simulink model "smart_irrigation_complete"  (R2026a)
settings: Solver=VariableStepAuto  StopTime=50
libraries: simulink x2

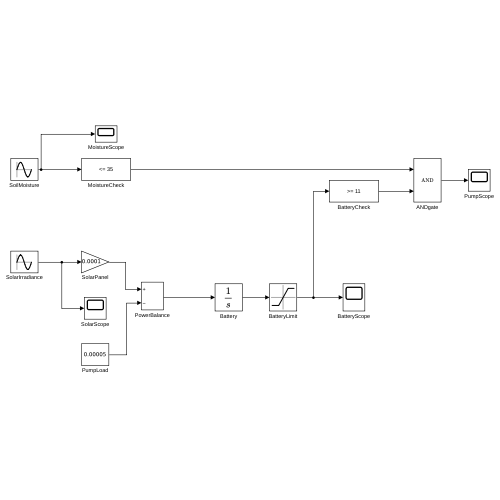
[thumbnail: Simulink's stored preview of the top-level diagram]
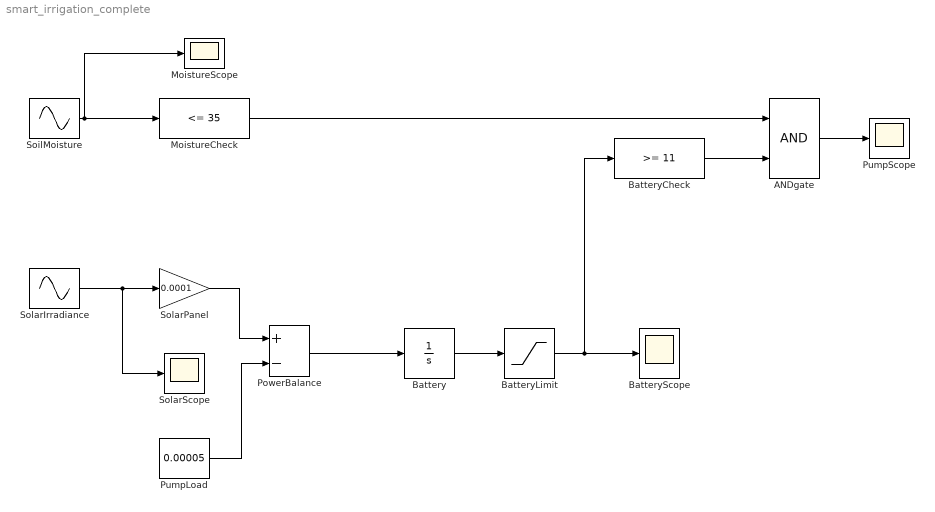
== system smart_irrigation_complete ==
  ANDgate : Logic  AllPortsSameDT=off  OutDataTypeStr=boolean
  Battery : Integrator  InitialCondition=12.4
  BatteryCheck : simulink/Logic and Bit Operations/Compare To Constant  relop=>=  const=11  OutDataTypeStr=boolean
  BatteryLimit : Saturate  UpperLimit=14.4  LowerLimit=10.5
  BatteryScope : Scope
  MoistureCheck : simulink/Logic and Bit Operations/Compare To Constant  relop=<=  const=35  OutDataTypeStr=boolean
  MoistureScope : Scope
  PowerBalance : Sum  Inputs=+-
  PumpLoad : Constant  Value=0.00005
  PumpScope : Scope
      settings: ActiveDisplayYMinimum=-0.12499999999999997  ActiveDisplayYMaximum=1.125
  SoilMoisture : Sin  Amplitude=20  Bias=45  Frequency=0.5  SampleTime=0
  SolarIrradiance : Sin  Amplitude=400  Bias=400  Frequency=0.2094  Phase=-1.5708  SampleTime=0
  SolarPanel : Gain  Gain=0.0001
  SolarScope : Scope
  wires:
  SoilMoisture/1 -> MoistureCheck/1, MoistureScope/1
  SolarIrradiance/1 -> SolarScope/1, SolarPanel/1
  SolarPanel/1 -> PowerBalance/1
  PumpLoad/1 -> PowerBalance/2
  PowerBalance/1 -> Battery/1
  Battery/1 -> BatteryLimit/1
  BatteryLimit/1 -> BatteryCheck/1, BatteryScope/1
  MoistureCheck/1 -> ANDgate/1
  BatteryCheck/1 -> ANDgate/2
  ANDgate/1 -> PumpScope/1
